simulink model "SpeedProfileTest"  (R2026b)
settings: Solver=FixedStepDiscrete  StopTime=profileTestCfg.Duration  FixedStep=profileCfg.Ts
PostLoadFcn:
  | addpath(fullfile(fileparts(get_param(bdroot,'FileName')),'..','build_process'));initialize_speed_profile_test(bdroot);
model workspace (MAT data in the model file):
  profileCfg.Ts = 5e-05
  profileCfg.Minimum = -15
  profileCfg.Maximum = 15
  profileCfg.RisingRate = 40
  profileCfg.FallingRate = 40
  profileCfg.RisingStep = 0.002
  profileCfg.FallingStep = 0.002
  profileTestCfg.Ts = 5e-05
  profileTestCfg.Duration = 0.5
  profileTestCfg.ReferenceInitial = 0
  profileTestCfg.Reference = 10
  profileTestCfg.CommandTime = 0.02
  profileTestCfg.ReverseReference = -10
  profileTestCfg.ReverseTime = 0.2
  profileTestCfg.DisableStart = 0.28
  profileTestCfg.DisableEnd = 0.32
  profileTestCfg.ResetTime = 0.4
  testStim.time = [0 5e-05 0.0001 0.00015 0.0002 0.00025 0.0003 0.00035 0.0004 0.00045 0.0005 0.00055 ... (10001 elements, 10001x1)]
  testStim.signals.values = [0 0 0 0 0 0 0 0 0 0 0 0 ... (30003 elements, 10001x3)]
  testStim.signals.dimensions = 3
libraries: MotionControl x1
settings Model: Creator=24322  LastModifiedBy=24322

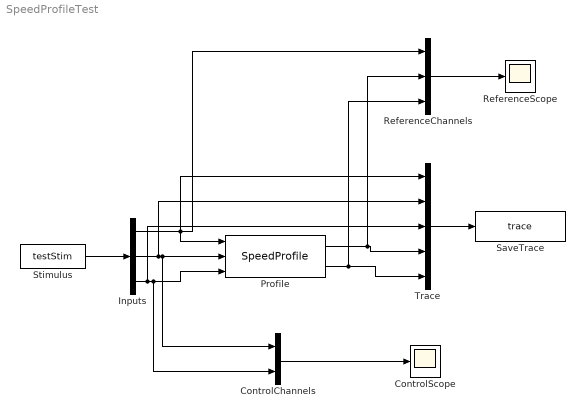
== system SpeedProfileTest ==
  ControlChannels : Mux  Inputs=2
  ControlScope : Scope
  Inputs : Demux  Outputs=3
  Profile : MotionControl/SpeedProfile  profileCfg=profileCfg
  ReferenceChannels : Mux  Inputs=3
  ReferenceScope : Scope
  SaveTrace : ToWorkspace  VariableName=trace  SaveFormat=Structure With Time  SampleTime=profileCfg.Ts
  Stimulus : FromWorkspace  VariableName=testStim  SampleTime=profileCfg.Ts  Interpolate=off  OutputAfterFinalValue=Holding final value
  Trace : Mux  Inputs=5
  wires:
  Inputs/3 -> ControlChannels/2, Profile/3, Trace/3
  Inputs/2 -> ControlChannels/1, Profile/2, Trace/2
  Profile/2 -> ReferenceChannels/3, Trace/5
  Profile/1 -> ReferenceChannels/2, Trace/4
  Inputs/1 -> Profile/1, ReferenceChannels/1, Trace/1
  ControlChannels/1 -> ControlScope/1
  ReferenceChannels/1 -> ReferenceScope/1
  Trace/1 -> SaveTrace/1
  Stimulus/1 -> Inputs/1
